simulink model "hrtf_v5_fest_olhead_ed1_38_L_2025a"  (R2025a)
settings: Solver=VariableStepAuto  StartTime=0.0  StopTime=10.0  RelTol=1e-3
values from neighbouring files (symbols this model uses):
  Alpha = [1 1 0.967796790113 -0.19525471365 0.941178659583 1.27759475775 0.157427422536 -0.232086624749 0.0400536246511 0.488732720219 -0.15013114138 -0.0870474720577 ... (18 elements, 2x9)]    [koeff_parameter_iir.mat]
  Beta = [1 1 4.50665299478 2.25254932437 11.1795102702 3.85997518129 18.0238230447 4.78060301042 20.7495830674 4.97041442912 17.1226318925 4.54493537547 ... (18 elements, 2x9)]    [koeff_parameter_iir.mat]
  Delay = [8966.24819844 7620.20448403]    [koeff_parameter_iir.mat]
  Gain = [4.7297619183 7.71004347236]    [koeff_parameter_iir.mat]
undefined symbols (not defined in the file or in its folder): dspblkCoreblockFVToolHelper, gcbh
settings Model: Creator=kucuk  LastModifiedBy=eoencue1

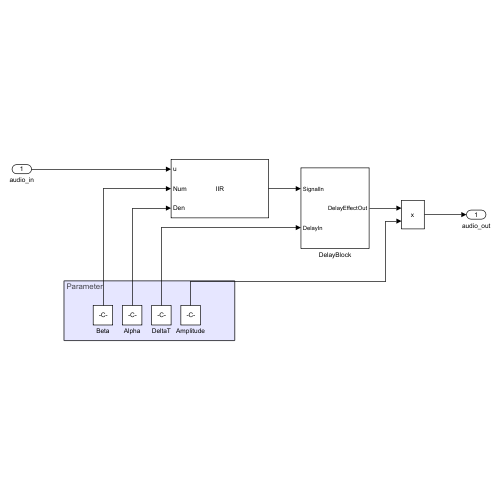
[thumbnail: Simulink's stored preview of the top-level diagram]
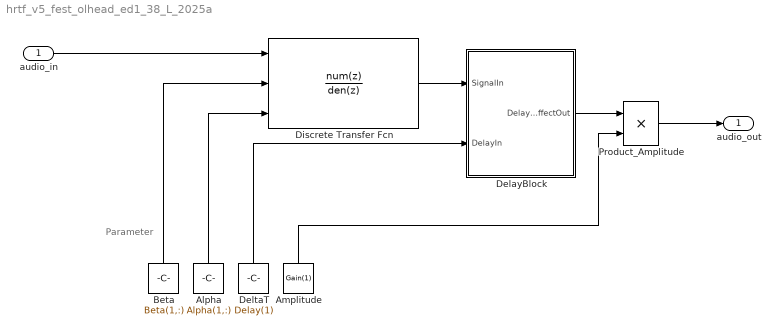
== system hrtf_v5_fest_olhead_ed1_38_L_2025a ==
  note: Parameter
  audio_in : Inport
  Alpha : Constant  Value=Alpha(1,:)
  Amplitude : Constant  Value=Gain(1)
  Beta : Constant  Value=Beta(1,:)
  DelayBlock : Subsystem
  DeltaT : Constant  Value=Delay(1)
  Discrete Transfer Fcn : DiscreteTransferFcn  LoadFcn=dspblkCoreblockFVToolHelper(gcbh,'load');  NumeratorSource=Input port  DenominatorSource=Input port  a0EqualsOne=on
      settings: CopyFcn=dspblkCoreblockFVToolHelper(gcbh,'copy');  DeleteFcn=dspblkCoreblockFVToolHelper(gcbh,'close');  ModelCloseFcn=dspblkCoreblockFVToolHelper(gcbh,'close');  PreSaveFcn=dspblkCoreblockFVToolHelper(gcbh,'presave');  PostSaveFcn=dspblkCoreblockFVToolHelper(gcbh,'postsave');  CloseFcn=dspblkCoreblockFVToolHelper(gcbh,'close');  InputPortMap=u0,p1,p3
  Product_Amplitude : Product
  audio_out : Outport
  wires:
  audio_in/1 -> Discrete Transfer Fcn/1
  Product_Amplitude/1 -> audio_out/1
  Beta/1 -> Discrete Transfer Fcn/2
  Amplitude/1 -> Product_Amplitude/2
  Alpha/1 -> Discrete Transfer Fcn/3
  Discrete Transfer Fcn/1 -> DelayBlock/1(SignalIn)
  DeltaT/1 -> DelayBlock/2(DelayIn)
  DelayBlock/1(DelayEffectOut) -> Product_Amplitude/1

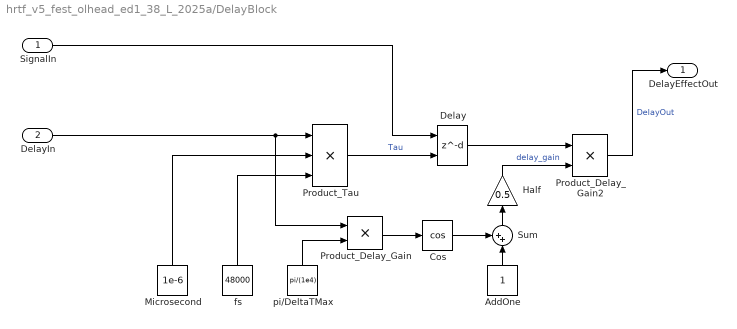
== system hrtf_v5_fest_olhead_ed1_38_L_2025a/DelayBlock ==
  SignalIn : Inport
  DelayIn : Inport  Port=2
  AddOne : Constant
  Cos : Trigonometry  Operator=cos
  Delay : Delay  DelayLengthSource=Input port  DelayLengthUpperLimit=10*48000*1e-3
      settings: InputPortMap=u0,p1
  Half : Gain  Gain=0.5
  Microsecond : Constant  Value=1e-6
  Product_Delay_Gain : Product
  Product_Delay_Gain2 : Product
  Product_Tau : Product  Inputs=3
  Sum : Sum  Inputs=++|
  fs : Constant  Value=48000
  pi/DeltaTMax : Constant  Value=pi/(1e4)
  DelayEffectOut : Outport
  wires:
  fs/1 -> Product_Tau/3
  Sum/1 -> Half/1
  pi/DeltaTMax/1 -> Product_Delay_Gain/2
  Delay/1 -> Product_Delay_Gain2/1
  Product_Tau/1 -> Delay/2  "Tau"
  Product_Delay_Gain/1 -> Cos/1
  DelayIn/1 -> Product_Delay_Gain/1, Product_Tau/1
  Microsecond/1 -> Product_Tau/2
  AddOne/1 -> Sum/2
  Half/1 -> Product_Delay_Gain2/2  "delay_gain"
  Cos/1 -> Sum/1
  Product_Delay_Gain2/1 -> DelayEffectOut/1  "DelayOut"
  SignalIn/1 -> Delay/1
